simulink model "windshear_pid_aircraft"  (R2019a)
settings: Solver=ode45  StartTime=0.0  StopTime=tstop  MaxStep=0.02  RelTol=1e-3
values from neighbouring files (symbols this model uses):
  Ah = 15    [windshear_params.m]
  Aw = 8    [windshear_params.m]
  dmax = deg2rad(25)    [windshear_params.m]
  hcmd = 0    [windshear_params.m]
  Kd = 0.8    [windshear_params.m]
  Kdh = 0.015    [windshear_params.m]
  Ki = 0.8    [windshear_params.m]
  Kih = 0.0006    [windshear_params.m]
  Kp = 2.0    (= 2)    [windshear_params.m]
  Kph = 0.006    [windshear_params.m]
  Mal = -6.0    (= -6)    [windshear_params.m]
  Md = 5.0    (= 5)    [windshear_params.m]
  Mq = -1.5    [windshear_params.m]
  Nf = 20    [windshear_params.m]
  Nfh = 10    [windshear_params.m]
  ShearOn = 1    [windshear_params.m]
  t0 = 20    [windshear_params.m]
  tau_act = 0.05    [windshear_params.m]
  tauV = 15    [windshear_params.m]
  theta_cmd_max = deg2rad(10)    [windshear_params.m]
  Tshear = 20    [windshear_params.m]
  V0 = 150    [windshear_params.m]
  Za = 1.0    (= 1)    [windshear_params.m]
libraries: simulink x2
settings Model: Creator=ABHI  LastModifiedBy=ABHI

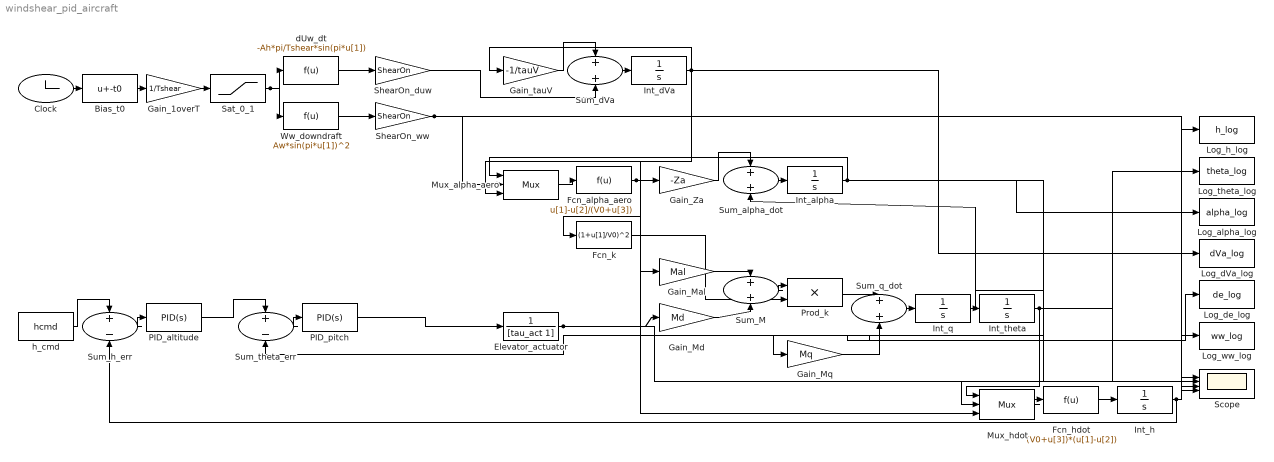
== system windshear_pid_aircraft ==
  Bias_t0 : Bias  Bias=-t0
  Clock : Clock
  Elevator_actuator : TransferFcn  Numerator=1  Denominator=[tau_act 1]
  Fcn_alpha_aero : Fcn  Expr=u[1]-u[2]/(V0+u[3])
  Fcn_hdot : Fcn  Expr=(V0+u[3])*(u[1]-u[2])
  Fcn_k : Fcn  Expr=(1+u[1]/V0)^2
  Gain_1overT : Gain  Gain=1/Tshear
  Gain_Mal : Gain  Gain=Mal
  Gain_Md : Gain  Gain=Md
  Gain_Mq : Gain  Gain=Mq
  Gain_Za : Gain  Gain=-Za
  Gain_tauV : Gain  Gain=-1/tauV
  Int_alpha : Integrator
  Int_dVa : Integrator
  Int_h : Integrator
  Int_q : Integrator
  Int_theta : Integrator
  Log_alpha_log : ToWorkspace  VariableName=alpha_log  SaveFormat=Timeseries  SampleTime=-1
  Log_dVa_log : ToWorkspace  VariableName=dVa_log  SaveFormat=Timeseries  SampleTime=-1
  Log_de_log : ToWorkspace  VariableName=de_log  SaveFormat=Timeseries  SampleTime=-1
  Log_h_log : ToWorkspace  VariableName=h_log  SaveFormat=Timeseries  SampleTime=-1
  Log_theta_log : ToWorkspace  VariableName=theta_log  SaveFormat=Timeseries  SampleTime=-1
  Log_ww_log : ToWorkspace  VariableName=ww_log  SaveFormat=Timeseries  SampleTime=-1
  Mux_alpha_aero : Mux  Inputs=3
  Mux_hdot : Mux  Inputs=3
  PID_altitude : simulink/Continuous/PID Controller  Controller=PID  Form=Parallel  TimeDomain=Continuous-time  SampleTime=-1  IntegratorMethod=Forward Euler  FilterMethod=Forward Euler  ControllerParametersSource=internal  P=Kph  I=Kih  D=Kdh  UseFilter=on  N=Nfh  TunerSelectOption=Transfer Function Based (PID Tuner App)  InitialConditionSource=internal  InitialConditionForIntegrator=0  InitialConditionForFilter=0  DifferentiatorICPrevScaledInput=0  ExternalReset=none  TrackingMode=off  Kt=1  LimitOutput=on  UpperSaturationLimit=theta_cmd_max  LowerSaturationLimit=-theta_cmd_max  LinearizeAsGain=on  AntiWindupMode=clamping  Kb=1  POutMin=[]  POutMax=[]  IOutMin=[]  IOutMax=[]  DOutMin=[]  DOutMax=[]  NOutMin=[]  NOutMax=[]  SumOutMin=[]  SumOutMax=[]  SaturationOutMin=[]  SaturationOutMax=[]  PParamMin=[]  PParamMax=[]  IParamMin=[]  IParamMax=[]  DParamMin=[]  DParamMax=[]  NParamMin=[]  NParamMax=[]  KbParamMin=[]  KbParamMax=[]  KtParamMin=[]  KtParamMax=[]  KbOutMin=[]  KbOutMax=[]  KtOutMin=[]  KtOutMax=[]  IntegratorOutMin=[]  IntegratorOutMax=[]  FilterOutMin=[]  FilterOutMax=[]  SumI1OutMin=[]  SumI1OutMax=[]  SumI2OutMin=[]  SumI2OutMax=[]  SumI3OutMin=[]  SumI3OutMax=[]  SumI4OutMin=[]  SumI4OutMax=[]  SumDOutMin=[]  SumDOutMax=[]  DifferentiatorOutMin=[]  DifferentiatorOutMax=[]  FilterDiffOutCoefMin=[]  FilterDiffOutCoefMax=[]  ReciprocalOutMin=[]  ReciprocalOutMax=[]  SumDenOutMin=[]  SumDenOutMax=[]  SumNumOutMin=[]  SumNumOutMax=[]  DivideOutMin=[]  DivideOutMax=[]  IntegratorContinuousStateAttributes=''  IntegratorStateMustResolveToSignalObject=off  IntegratorRTWStateStorageClass=Auto  FilterContinuousStateAttributes=''  FilterStateMustResolveToSignalObject=off  FilterRTWStateStorageClass=Auto  ParallelPVariant=InternalParameters  IdealPVariant=Disabled  IVariant=InternalParameters  DVariant=InternalParameters  IntegratorVariant=Continuous  SatVariant=Enabled  AWVariant=ContClampingParallel  PCopyVariant=Disabled  TRVariant=Disabled  FdbkBlocksVariant=Forward  IdealPFdbkVariant=Disabled  SatFdbkVariant=Disabled  DerivativeFilterVariant=ContFilter  NVariant=InternalParameters  NCopyVariant=Disabled  FilterICVariant=InternalICsFilter  IntegratorICVariant=InternalICs  ExternalResetVariant=Disabled  TRSumVariant=Passthrough  SumFdbkVariant=Disabled  SumVariant=Sum_PID
  PID_pitch : simulink/Continuous/PID Controller  Controller=PID  Form=Parallel  TimeDomain=Continuous-time  SampleTime=-1  IntegratorMethod=Forward Euler  FilterMethod=Forward Euler  ControllerParametersSource=internal  P=Kp  I=Ki  D=Kd  UseFilter=on  N=Nf  TunerSelectOption=Transfer Function Based (PID Tuner App)  InitialConditionSource=internal  InitialConditionForIntegrator=0  InitialConditionForFilter=0  DifferentiatorICPrevScaledInput=0  ExternalReset=none  TrackingMode=off  Kt=1  LimitOutput=on  UpperSaturationLimit=dmax  LowerSaturationLimit=-dmax  LinearizeAsGain=on  AntiWindupMode=clamping  Kb=1  POutMin=[]  POutMax=[]  IOutMin=[]  IOutMax=[]  DOutMin=[]  DOutMax=[]  NOutMin=[]  NOutMax=[]  SumOutMin=[]  SumOutMax=[]  SaturationOutMin=[]  SaturationOutMax=[]  PParamMin=[]  PParamMax=[]  IParamMin=[]  IParamMax=[]  DParamMin=[]  DParamMax=[]  NParamMin=[]  NParamMax=[]  KbParamMin=[]  KbParamMax=[]  KtParamMin=[]  KtParamMax=[]  KbOutMin=[]  KbOutMax=[]  KtOutMin=[]  KtOutMax=[]  IntegratorOutMin=[]  IntegratorOutMax=[]  FilterOutMin=[]  FilterOutMax=[]  SumI1OutMin=[]  SumI1OutMax=[]  SumI2OutMin=[]  SumI2OutMax=[]  SumI3OutMin=[]  SumI3OutMax=[]  SumI4OutMin=[]  SumI4OutMax=[]  SumDOutMin=[]  SumDOutMax=[]  DifferentiatorOutMin=[]  DifferentiatorOutMax=[]  FilterDiffOutCoefMin=[]  FilterDiffOutCoefMax=[]  ReciprocalOutMin=[]  ReciprocalOutMax=[]  SumDenOutMin=[]  SumDenOutMax=[]  SumNumOutMin=[]  SumNumOutMax=[]  DivideOutMin=[]  DivideOutMax=[]  IntegratorContinuousStateAttributes=''  IntegratorStateMustResolveToSignalObject=off  IntegratorRTWStateStorageClass=Auto  FilterContinuousStateAttributes=''  FilterStateMustResolveToSignalObject=off  FilterRTWStateStorageClass=Auto  ParallelPVariant=InternalParameters  IdealPVariant=Disabled  IVariant=InternalParameters  DVariant=InternalParameters  IntegratorVariant=Continuous  SatVariant=Enabled  AWVariant=ContClampingParallel  PCopyVariant=Disabled  TRVariant=Disabled  FdbkBlocksVariant=Forward  IdealPFdbkVariant=Disabled  SatFdbkVariant=Disabled  DerivativeFilterVariant=ContFilter  NVariant=InternalParameters  NCopyVariant=Disabled  FilterICVariant=InternalICsFilter  IntegratorICVariant=InternalICs  ExternalResetVariant=Disabled  TRSumVariant=Passthrough  SumFdbkVariant=Disabled  SumVariant=Sum_PID
  Prod_k : Product
  Sat_0_1 : Saturate  UpperLimit=1  LowerLimit=0
  Scope : Scope  NumInputPorts=4
  ShearOn_duw : Gain  Gain=ShearOn
  ShearOn_ww : Gain  Gain=ShearOn
  Sum_M : Sum
  Sum_alpha_dot : Sum
  Sum_dVa : Sum
  Sum_h_err : Sum  Inputs=+-
  Sum_q_dot : Sum
  Sum_theta_err : Sum  Inputs=+-
  Ww_downdraft : Fcn  Expr=Aw*sin(pi*u[1])^2
  dUw_dt : Fcn  Expr=-Ah*pi/Tshear*sin(pi*u[1])
  h_cmd : Constant  Value=hcmd
  wires:
  Clock/1 -> Bias_t0/1
  Bias_t0/1 -> Gain_1overT/1
  Gain_1overT/1 -> Sat_0_1/1
  Sat_0_1/1 -> dUw_dt/1, Ww_downdraft/1
  dUw_dt/1 -> ShearOn_duw/1
  Ww_downdraft/1 -> ShearOn_ww/1
  Int_dVa/1 -> Gain_tauV/1, Mux_alpha_aero/3, Fcn_k/1, Mux_hdot/3, Log_dVa_log/1
  Gain_tauV/1 -> Sum_dVa/1
  ShearOn_duw/1 -> Sum_dVa/2
  Sum_dVa/1 -> Int_dVa/1
  Int_alpha/1 -> Mux_alpha_aero/1, Mux_hdot/2, Log_alpha_log/1
  ShearOn_ww/1 -> Mux_alpha_aero/2, Log_ww_log/1, Scope/4
  Mux_alpha_aero/1 -> Fcn_alpha_aero/1
  Fcn_alpha_aero/1 -> Gain_Za/1, Gain_Mal/1
  Gain_Za/1 -> Sum_alpha_dot/1
  Int_q/1 -> Sum_alpha_dot/2, Gain_Mq/1, Int_theta/1
  Sum_alpha_dot/1 -> Int_alpha/1
  Gain_Mal/1 -> Sum_M/1
  Gain_Md/1 -> Sum_M/2
  Sum_M/1 -> Prod_k/1
  Fcn_k/1 -> Prod_k/2
  Prod_k/1 -> Sum_q_dot/1
  Gain_Mq/1 -> Sum_q_dot/2
  Sum_q_dot/1 -> Int_q/1
  Int_theta/1 -> Mux_hdot/1, Sum_theta_err/2, Log_theta_log/1, Scope/2
  Mux_hdot/1 -> Fcn_hdot/1
  Fcn_hdot/1 -> Int_h/1
  Elevator_actuator/1 -> Gain_Md/1, Log_de_log/1, Scope/3
  h_cmd/1 -> Sum_h_err/1
  Int_h/1 -> Sum_h_err/2, Log_h_log/1, Scope/1
  Sum_h_err/1 -> PID_altitude/1
  PID_altitude/1 -> Sum_theta_err/1
  Sum_theta_err/1 -> PID_pitch/1
  PID_pitch/1 -> Elevator_actuator/1
